simulink model "lab12"  (R2025b)
settings: Solver=VariableStepAuto  StartTime=0.0  StopTime=10.0  RelTol=1e-3
undefined symbols (not defined in the file): A, b, denW, gamma, K, numW
settings Model: Creator=Nickolay  LastModifiedBy=Nickolay

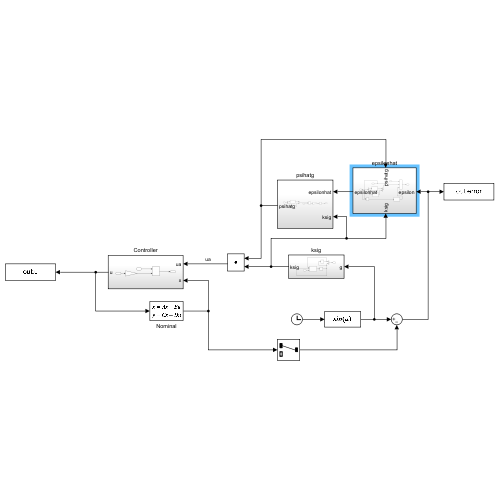
[thumbnail: Simulink's stored preview of the top-level diagram]
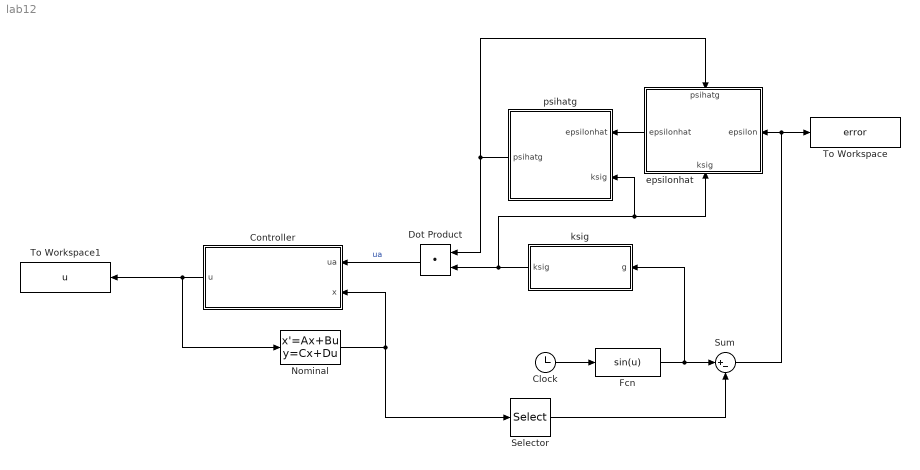
== system lab12 ==
  Clock : Clock
  Controller : Subsystem
  Dot Product : DotProduct  OutDataTypeStr=Inherit: Inherit via internal rule
  Fcn : Fcn  Expr=sin(u)
  Nominal : StateSpace  A=A  B=b  C=eye(2)  D=zeros(2,1)  InitialCondition=0
  Selector : Selector  InputPortWidth=2  IndexOptions=Index vector (dialog)  Indices=1  OutputSizes=1
  Sum : Sum  Inputs=|+-
  To Workspace : ToWorkspace  VariableName=error  SaveFormat=Timeseries  SampleTime=-1
  To Workspace1 : ToWorkspace  VariableName=u  SaveFormat=Timeseries  SampleTime=-1
  epsilonhat : Subsystem
      settings: PortSchema="{\"entries\":[{\"content\":{\"sides\":[{\"content\":{\"connectorIds\":[\"In1\"]},\"type\":\"ConnectorPlacement.EquallySpacedRectSide\",\"uuid\":\"f6a236b5-2f9f-4fb8-9e71-5a9dd2d5c3e7\"},{\"content\":{\"connectorIds\":[\"Out1\"],\"side\":\"RIGHT\"},\"type\":\"ConnectorPlacement.EquallySpacedRectSide\",\"uuid\":\"354f96b2-fadf-4299-baeb-f66ebfe4292e\"},{\"content\":{\"connectorIds\":[\"In2\"],\"side\":\"TOP\"},\"type\":\"ConnectorPlacement.EquallySpacedRectSide\",\"uuid\":\"004cc3ef-e854-435e-a531-55bfb8f067e1\"},{\"content\":{\"connectorIds\":[\"In3\"],\"side\":\"BOTTOM\"},\"type\":\"ConnectorPlacement.EquallySpacedRectSide\",\"uuid\":\"09c3f0f0-cd43-4fb8-9dee-bea826c0b5f1\"}]},\"type\":\"ConnectorPlacement.EquallySpacedConnector\",\"uuid\":\"69a88c44-6962-4886-992d-ed9ea791b010\"}],\"packageUris\":[\"http://schema.mathworks.com/mf0/Connector/R2020b\"],\"version\":\"1.0\"}"
  ksig : Subsystem
  psihatg : Subsystem
  wires:
  Nominal/1 -> Selector/1, Controller/2(x)
  Controller/1(u) -> Nominal/1, To Workspace1/1
  ksig/1(ksig) -> epsilonhat/3(ksig), psihatg/2(ksig), Dot Product/2
  psihatg/1(psihatg) -> epsilonhat/2(psihatg), Dot Product/1
  Dot Product/1 -> Controller/1(ua)  "ua"
  Sum/1 -> epsilonhat/1(epsilon), To Workspace/1
  epsilonhat/1(epsilonhat) -> psihatg/1(epsilonhat)
  Fcn/1 -> Sum/1, ksig/1(g)
  Clock/1 -> Fcn/1
  Selector/1 -> Sum/2

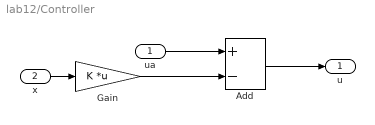
== system lab12/Controller ==
  ua : Inport
  x : Inport  Port=2
  Add : Sum  Inputs=+-
  Gain : Gain  Gain=K  Multiplication=Matrix(K*u) (u vector)
  u : Outport
  wires:
  ua/1 -> Add/1
  Add/1 -> u/1
  x/1 -> Gain/1
  Gain/1 -> Add/2

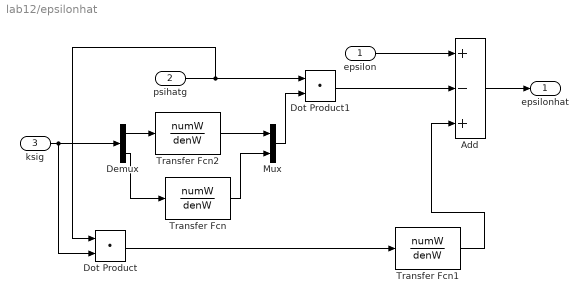
== system lab12/epsilonhat ==
  epsilon : Inport
  psihatg : Inport  Port=2
  ksig : Inport  Port=3
  Add : Sum  Inputs=+-+
  Demux : Demux  Outputs=2
  Dot Product : DotProduct  OutDataTypeStr=Inherit: Inherit via internal rule
  Dot Product1 : DotProduct  OutDataTypeStr=Inherit: Inherit via internal rule
  Mux : Mux  Inputs=2
  Transfer Fcn : TransferFcn  Numerator=numW  Denominator=denW
  Transfer Fcn1 : TransferFcn  Numerator=numW  Denominator=denW
  Transfer Fcn2 : TransferFcn  Numerator=numW  Denominator=denW
  epsilonhat : Outport
  wires:
  Add/1 -> epsilonhat/1
  epsilon/1 -> Add/1
  ksig/1 -> Dot Product/2, Demux/1
  Dot Product1/1 -> Add/2
  psihatg/1 -> Dot Product1/1, Dot Product/1
  Demux/2 -> Transfer Fcn/1
  Transfer Fcn/1 -> Mux/2
  Demux/1 -> Transfer Fcn2/1
  Transfer Fcn2/1 -> Mux/1
  Mux/1 -> Dot Product1/2
  Transfer Fcn1/1 -> Add/3
  Dot Product/1 -> Transfer Fcn1/1

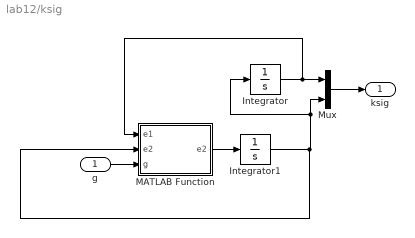
== system lab12/ksig ==
  g : Inport
  Integrator : Integrator
  Integrator1 : Integrator
  MATLAB Function : MATLAB Function  TreatAsAtomicUnit=on
  Mux : Mux  Inputs=2
  ksig : Outport  PortDimensions=2
  wires:
  Mux/1 -> ksig/1
  Integrator/1 -> MATLAB Function/1(e1), Mux/1
  g/1 -> MATLAB Function/3(g)
  MATLAB Function/1(e2) -> Integrator1/1
  Integrator1/1 -> MATLAB Function/2("e2 "), Mux/2, Integrator/1

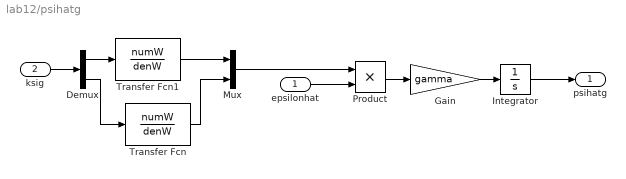
== system lab12/psihatg ==
  epsilonhat : Inport
  ksig : Inport  Port=2
  Demux : Demux  Outputs=2
  Gain : Gain  Gain=gamma
  Integrator : Integrator  InitialCondition=[0; 0]
  Mux : Mux  Inputs=2
  Product : Product
  Transfer Fcn : TransferFcn  Numerator=numW  Denominator=denW
  Transfer Fcn1 : TransferFcn  Numerator=numW  Denominator=denW
  psihatg : Outport  PortDimensions=2
  wires:
  Integrator/1 -> psihatg/1
  epsilonhat/1 -> Product/2
  Transfer Fcn/1 -> Mux/2
  Product/1 -> Gain/1
  Gain/1 -> Integrator/1
  ksig/1 -> Demux/1
  Demux/1 -> Transfer Fcn1/1
  Demux/2 -> Transfer Fcn/1
  Transfer Fcn1/1 -> Mux/1
  Mux/1 -> Product/1

== matlab function lab12/ksig/MATLAB Function ==
  data: e1 input; e2 output; e2 input; g input
function e2 = fcn(e1,e2,g)
e2 = -0.16*e1-0.8*e2+g;
